simulink model "adc_behavioral"  (R2026a)
settings: Solver=FixedStepDiscrete  StartTime=0  StopTime=4095  FixedStep=1
model workspace (MAT data in the model file):
  C : object (value not decoded)
  d1_signal = [0 1 2 3 4 5 6 7 8 9 10 11 ... (8192 elements, 4096x2)]
  d2_signal = [0 1 2 3 4 5 6 7 8 9 10 11 ... (8192 elements, 4096x2)]
  n_signal = [0 1 2 3 4 5 6 7 8 9 10 11 ... (8192 elements, 4096x2)]
  x_signal = [0 1 2 3 4 5 6 7 8 9 10 11 ... (8192 elements, 4096x2)]
values from neighbouring files (symbols this model uses):
  C = entry.parameters    [adc_load_case.m]    (also in audit_adc_model.m = evalin(workspace,'C'))
(part 2 of 2)

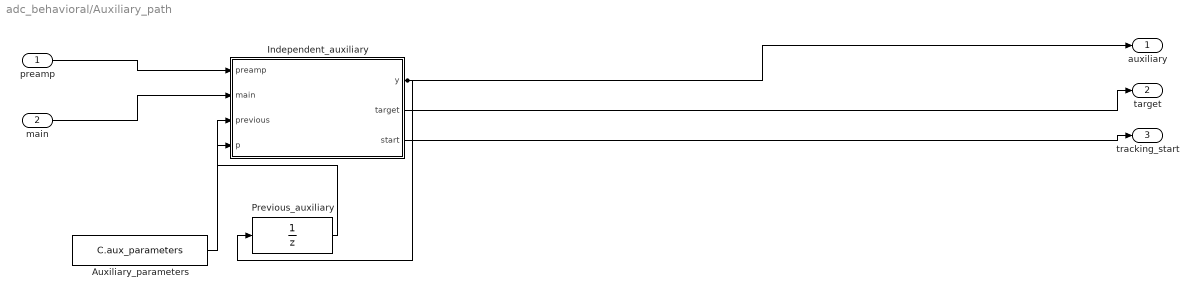
== system adc_behavioral/Auxiliary_path ==
  preamp : Inport
  main : Inport  Port=2
  Auxiliary_parameters : Constant  Value=C.aux_parameters  SampleTime=1
  Independent_auxiliary : MATLAB Function  TreatAsAtomicUnit=on
  Previous_auxiliary : UnitDelay  InitialCondition=C.initial_analog(2)
  auxiliary : Outport
  target : Outport  Port=2
  tracking_start : Outport  Port=3
  wires:
  preamp/1 -> Independent_auxiliary/1(preamp)
  main/1 -> Independent_auxiliary/2(main)
  Previous_auxiliary/1 -> Independent_auxiliary/3(previous)
  Auxiliary_parameters/1 -> Independent_auxiliary/4(p)
  Independent_auxiliary/1(y) -> Previous_auxiliary/1, auxiliary/1
  Independent_auxiliary/2(target) -> target/1
  Independent_auxiliary/3(start) -> tracking_start/1

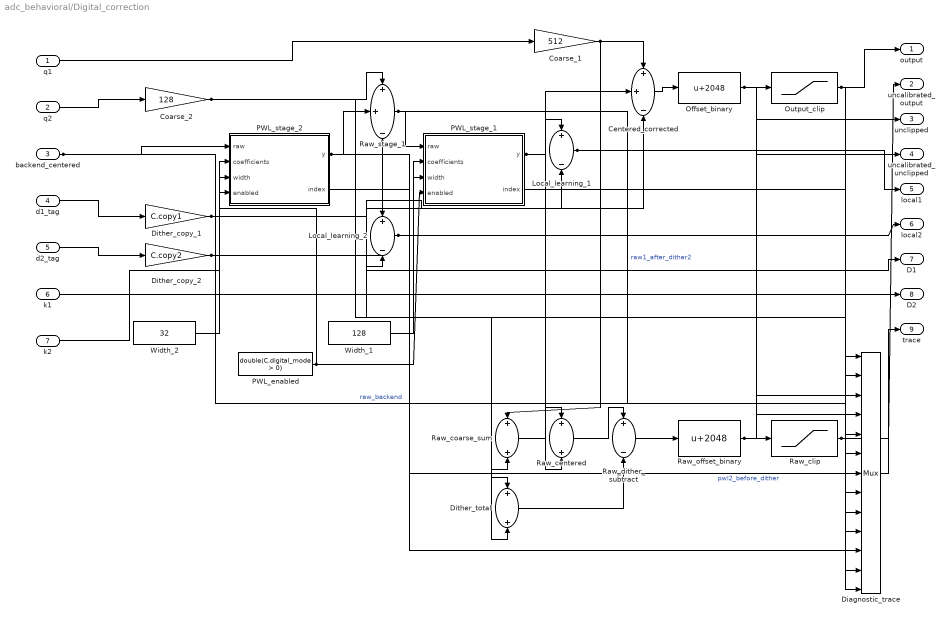
== system adc_behavioral/Digital_correction ==
  q1 : Inport
  q2 : Inport  Port=2
  backend_centered : Inport  Port=3
  d1_tag : Inport  Port=4
  d2_tag : Inport  Port=5
  k1 : Inport  Port=6
  k2 : Inport  Port=7
  Centered_corrected : Sum  Inputs=++-
  Coarse_1 : Gain  Gain=512
  Coarse_2 : Gain  Gain=128
  Diagnostic_trace : Mux  Inputs=13
  Dither_copy_1 : Gain  Gain=C.copy1
  Dither_copy_2 : Gain  Gain=C.copy2
  Dither_total : Sum
  Local_learning_1 : Sum  Inputs=+-
  Local_learning_2 : Sum  Inputs=+-
  Offset_binary : Bias  Bias=2048  SaturateOnIntegerOverflow=off
  Output_clip : Saturate  UpperLimit=4095  LowerLimit=0
  PWL_enabled : Constant  Value=double(C.digital_mode > 0)  SampleTime=1
  PWL_stage_1 : MATLAB Function  TreatAsAtomicUnit=on
  PWL_stage_2 : MATLAB Function  TreatAsAtomicUnit=on
  Raw_centered : Sum
  Raw_clip : Saturate  UpperLimit=4095  LowerLimit=0
  Raw_coarse_sum : Sum
  Raw_dither_subtract : Sum  Inputs=+-
  Raw_offset_binary : Bias  Bias=2048  SaturateOnIntegerOverflow=off
  Raw_stage_1 : Sum  Inputs=++-
  Width_1 : Constant  Value=128  SampleTime=1
  Width_2 : Constant  Value=32  SampleTime=1
  output : Outport
  uncalibrated_output : Outport  Port=2
  unclipped : Outport  Port=3
  uncalibrated_unclipped : Outport  Port=4
  local1 : Outport  Port=5
  local2 : Outport  Port=6
  D1 : Outport  Port=7
  D2 : Outport  Port=8
  trace : Outport  Port=9
  wires:
  d1_tag/1 -> Dither_copy_1/1
  d2_tag/1 -> Dither_copy_2/1
  q1/1 -> Coarse_1/1
  q2/1 -> Coarse_2/1
  backend_centered/1 -> PWL_stage_2/1(raw), Raw_centered/2  "raw_backend"
  k2/1 -> PWL_stage_2/2(coefficients)
  Width_2/1 -> PWL_stage_2/3(width)
  PWL_enabled/1 -> PWL_stage_2/4(enabled), PWL_stage_1/4(enabled)
  Coarse_2/1 -> Raw_stage_1/1, Raw_coarse_sum/2
  PWL_stage_2/1(y) -> Raw_stage_1/2, Local_learning_2/1, Diagnostic_trace/7  "pwl2_before_dither"
  Dither_copy_2/1 -> Raw_stage_1/3, Local_learning_2/2, Dither_total/2, D2/1, Diagnostic_trace/13
  Raw_stage_1/1 -> PWL_stage_1/1(raw), Diagnostic_trace/5  "raw1_after_dither2"
  k1/1 -> PWL_stage_1/2(coefficients)
  Width_1/1 -> PWL_stage_1/3(width)
  PWL_stage_1/1(y) -> Local_learning_1/1, Centered_corrected/2, Diagnostic_trace/6
  Dither_copy_1/1 -> Local_learning_1/2, Centered_corrected/3, Dither_total/1, D1/1, Diagnostic_trace/12
  Coarse_1/1 -> Centered_corrected/1, Raw_coarse_sum/1
  Centered_corrected/1 -> Offset_binary/1
  Offset_binary/1 -> Output_clip/1, unclipped/1, Diagnostic_trace/3
  Raw_coarse_sum/1 -> Raw_centered/1
  Raw_centered/1 -> Raw_dither_subtract/1
  Dither_total/1 -> Raw_dither_subtract/2
  Raw_dither_subtract/1 -> Raw_offset_binary/1
  Raw_offset_binary/1 -> Raw_clip/1, uncalibrated_unclipped/1, Diagnostic_trace/4
  Output_clip/1 -> output/1, Diagnostic_trace/1
  Raw_clip/1 -> uncalibrated_output/1, Diagnostic_trace/2
  Local_learning_1/1 -> local1/1, Diagnostic_trace/8
  Local_learning_2/1 -> local2/1, Diagnostic_trace/9
  PWL_stage_1/2(index) -> Diagnostic_trace/10
  PWL_stage_2/2(index) -> Diagnostic_trace/11
  Diagnostic_trace/1 -> trace/1

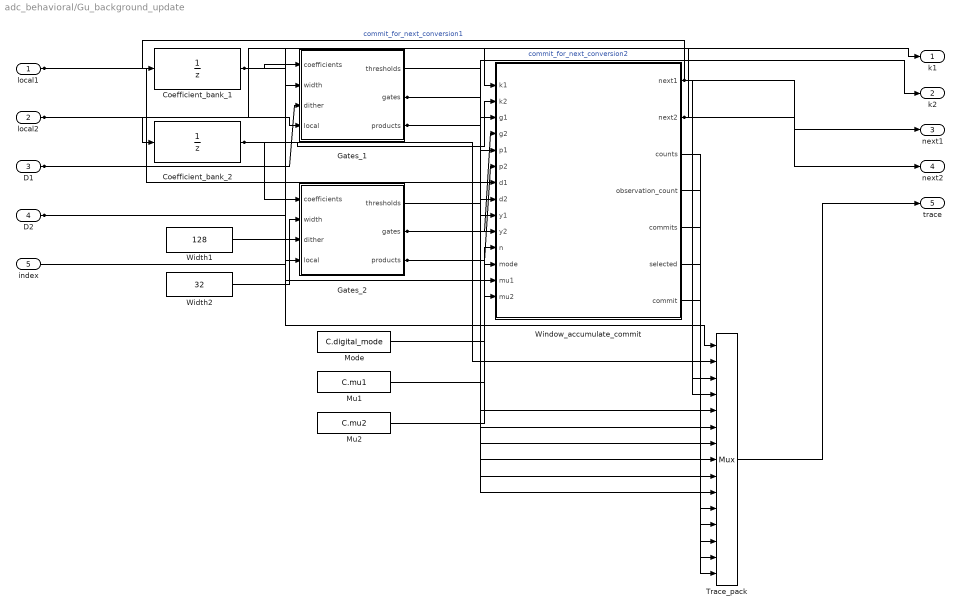
== system adc_behavioral/Gu_background_update ==
  local1 : Inport
  local2 : Inport  Port=2
  D1 : Inport  Port=3
  D2 : Inport  Port=4
  index : Inport  Port=5
  Coefficient_bank_1 : UnitDelay  InitialCondition=C.initial1
  Coefficient_bank_2 : UnitDelay  InitialCondition=C.initial2
  Gates_1 : MATLAB Function  TreatAsAtomicUnit=on
  Gates_2 : MATLAB Function  TreatAsAtomicUnit=on
  Mode : Constant  Value=C.digital_mode  SampleTime=1
  Mu1 : Constant  Value=C.mu1  SampleTime=1
  Mu2 : Constant  Value=C.mu2  SampleTime=1
  Trace_pack : Mux  Inputs=15
  Width1 : Constant  Value=128  SampleTime=1
  Width2 : Constant  Value=32  SampleTime=1
  Window_accumulate_commit : MATLAB Function  TreatAsAtomicUnit=on
  k1 : Outport
  k2 : Outport  Port=2
  next1 : Outport  Port=3
  next2 : Outport  Port=4
  trace : Outport  Port=5
  wires:
  Coefficient_bank_1/1 -> Gates_1/1(coefficients), Window_accumulate_commit/1(k1), k1/1, Trace_pack/1
  Coefficient_bank_2/1 -> Gates_2/1(coefficients), Window_accumulate_commit/2(k2), k2/1, Trace_pack/2
  Width1/1 -> Gates_1/2(width)
  Width2/1 -> Gates_2/2(width)
  D1/1 -> Gates_1/3(dither), Window_accumulate_commit/7(d1)
  D2/1 -> Gates_2/3(dither), Window_accumulate_commit/8(d2)
  local1/1 -> Gates_1/4(local), Window_accumulate_commit/9(y1)
  local2/1 -> Gates_2/4(local), Window_accumulate_commit/10(y2)
  Gates_1/2(gates) -> Window_accumulate_commit/3(g1), Trace_pack/7
  Gates_2/2(gates) -> Window_accumulate_commit/4(g2), Trace_pack/8
  Gates_1/3(products) -> Window_accumulate_commit/5(p1), Trace_pack/9
  Gates_2/3(products) -> Window_accumulate_commit/6(p2), Trace_pack/10
  index/1 -> Window_accumulate_commit/11(n)
  Mode/1 -> Window_accumulate_commit/12(mode)
  Mu1/1 -> Window_accumulate_commit/13(mu1)
  Mu2/1 -> Window_accumulate_commit/14(mu2)
  Window_accumulate_commit/1(next1) -> Coefficient_bank_1/1, next1/1, Trace_pack/3  "commit_for_next_conversion1"
  Window_accumulate_commit/2(next2) -> Coefficient_bank_2/1, next2/1, Trace_pack/4  "commit_for_next_conversion2"
  Gates_1/1(thresholds) -> Trace_pack/5
  Gates_2/1(thresholds) -> Trace_pack/6
  Window_accumulate_commit/3(counts) -> Trace_pack/11
  Window_accumulate_commit/4(observation_count) -> Trace_pack/12
  Window_accumulate_commit/5(commits) -> Trace_pack/13
  Window_accumulate_commit/6(selected) -> Trace_pack/14
  Window_accumulate_commit/7(commit) -> Trace_pack/15
  Trace_pack/1 -> trace/1

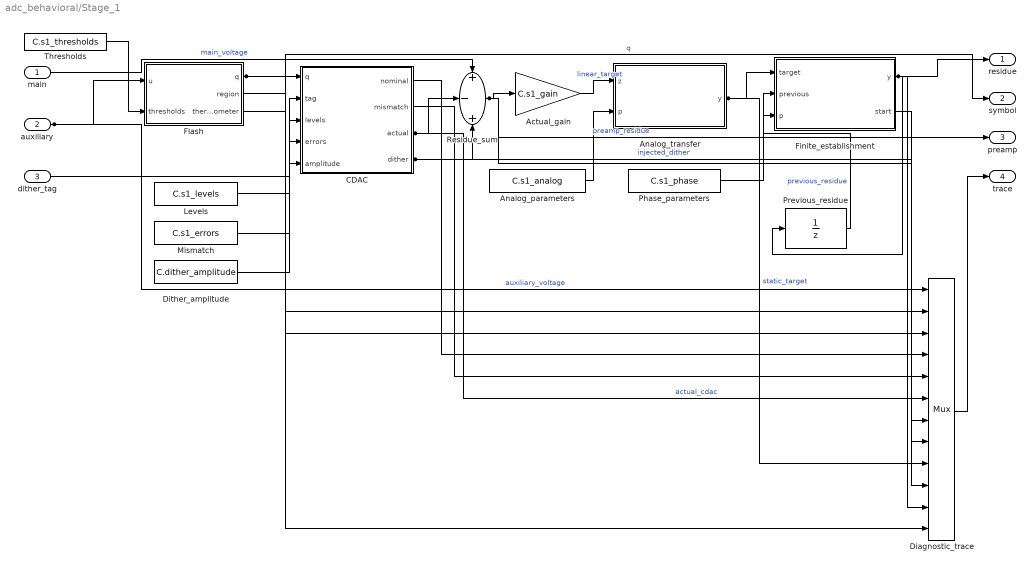
== system adc_behavioral/Stage_1 ==
  main : Inport
  auxiliary : Inport  Port=2
  dither_tag : Inport  Port=3
  Actual_gain : Gain  Gain=C.s1_gain
  Analog_parameters : Constant  Value=C.s1_analog  SampleTime=1
  Analog_transfer : MATLAB Function  TreatAsAtomicUnit=on
  CDAC : MATLAB Function  TreatAsAtomicUnit=on
  Diagnostic_trace : Mux  Inputs=12
  Dither_amplitude : Constant  Value=C.dither_amplitude  SampleTime=1
  Finite_establishment : MATLAB Function  TreatAsAtomicUnit=on
  Flash : MATLAB Function  TreatAsAtomicUnit=on
  Levels : Constant  Value=C.s1_levels  SampleTime=1
  Mismatch : Constant  Value=C.s1_errors  SampleTime=1
  Phase_parameters : Constant  Value=C.s1_phase  SampleTime=1
  Previous_residue : UnitDelay  InitialCondition=C.initial_analog(1)
  Residue_sum : Sum  Inputs=+-+
  Thresholds : Constant  Value=C.s1_thresholds  SampleTime=1
  residue : Outport
  symbol : Outport  Port=2
  preamp : Outport  Port=3
  trace : Outport  Port=4
  wires:
  auxiliary/1 -> Flash/1(u), Diagnostic_trace/1  "auxiliary_voltage"
  Thresholds/1 -> Flash/2(thresholds)
  Flash/1(q) -> CDAC/1(q), symbol/1, Diagnostic_trace/2  "q"
  dither_tag/1 -> CDAC/2(tag)
  Levels/1 -> CDAC/3(levels)
  Mismatch/1 -> CDAC/4(errors)
  Dither_amplitude/1 -> CDAC/5(amplitude)
  main/1 -> Residue_sum/1  "main_voltage"
  CDAC/3(actual) -> Residue_sum/2, Diagnostic_trace/6  "actual_cdac"
  CDAC/4(dither) -> Residue_sum/3, Diagnostic_trace/7  "injected_dither"
  Residue_sum/1 -> Actual_gain/1, preamp/1, Diagnostic_trace/8  "preamp_residue"
  Actual_gain/1 -> Analog_transfer/1(z)  "linear_target"
  Analog_parameters/1 -> Analog_transfer/2(p)
  Analog_transfer/1(y) -> Finite_establishment/1(target), Diagnostic_trace/9  "static_target"
  Previous_residue/1 -> Finite_establishment/2(previous)  "previous_residue"
  Phase_parameters/1 -> Finite_establishment/3(p)
  Finite_establishment/1(y) -> Previous_residue/1, residue/1, Diagnostic_trace/11
  Flash/2(region) -> Diagnostic_trace/3
  CDAC/1(nominal) -> Diagnostic_trace/4
  CDAC/2(mismatch) -> Diagnostic_trace/5
  Finite_establishment/2(start) -> Diagnostic_trace/10
  Flash/3(thermometer) -> Diagnostic_trace/12
  Diagnostic_trace/1 -> trace/1

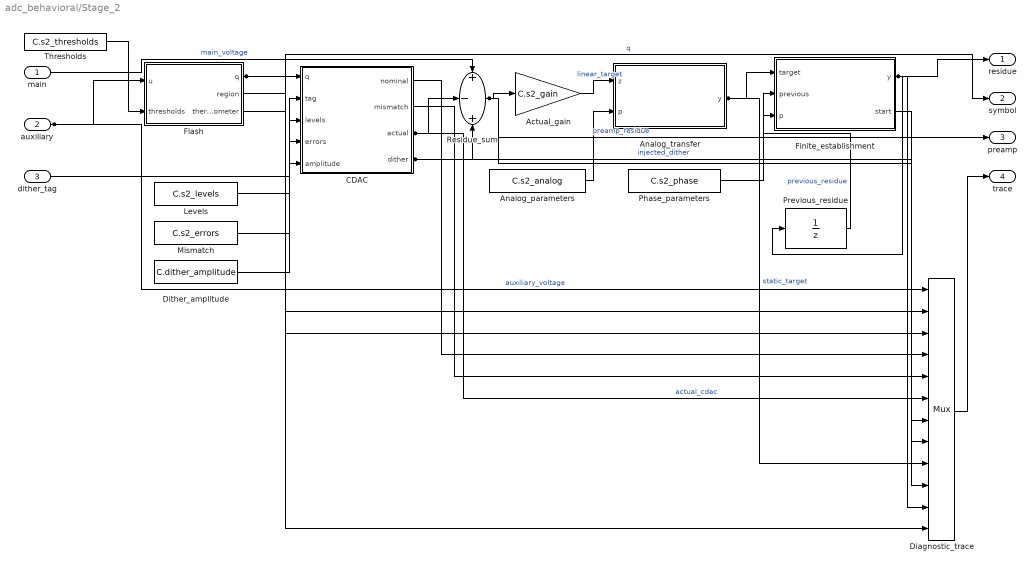
== system adc_behavioral/Stage_2 ==
  main : Inport
  auxiliary : Inport  Port=2
  dither_tag : Inport  Port=3
  Actual_gain : Gain  Gain=C.s2_gain
  Analog_parameters : Constant  Value=C.s2_analog  SampleTime=1
  Analog_transfer : MATLAB Function  TreatAsAtomicUnit=on
  CDAC : MATLAB Function  TreatAsAtomicUnit=on
  Diagnostic_trace : Mux  Inputs=12
  Dither_amplitude : Constant  Value=C.dither_amplitude  SampleTime=1
  Finite_establishment : MATLAB Function  TreatAsAtomicUnit=on
  Flash : MATLAB Function  TreatAsAtomicUnit=on
  Levels : Constant  Value=C.s2_levels  SampleTime=1
  Mismatch : Constant  Value=C.s2_errors  SampleTime=1
  Phase_parameters : Constant  Value=C.s2_phase  SampleTime=1
  Previous_residue : UnitDelay  InitialCondition=C.initial_analog(3)
  Residue_sum : Sum  Inputs=+-+
  Thresholds : Constant  Value=C.s2_thresholds  SampleTime=1
  residue : Outport
  symbol : Outport  Port=2
  preamp : Outport  Port=3
  trace : Outport  Port=4
  wires:
  auxiliary/1 -> Flash/1(u), Diagnostic_trace/1  "auxiliary_voltage"
  Thresholds/1 -> Flash/2(thresholds)
  Flash/1(q) -> CDAC/1(q), symbol/1, Diagnostic_trace/2  "q"
  dither_tag/1 -> CDAC/2(tag)
  Levels/1 -> CDAC/3(levels)
  Mismatch/1 -> CDAC/4(errors)
  Dither_amplitude/1 -> CDAC/5(amplitude)
  main/1 -> Residue_sum/1  "main_voltage"
  CDAC/3(actual) -> Residue_sum/2, Diagnostic_trace/6  "actual_cdac"
  CDAC/4(dither) -> Residue_sum/3, Diagnostic_trace/7  "injected_dither"
  Residue_sum/1 -> Actual_gain/1, preamp/1, Diagnostic_trace/8  "preamp_residue"
  Actual_gain/1 -> Analog_transfer/1(z)  "linear_target"
  Analog_parameters/1 -> Analog_transfer/2(p)
  Analog_transfer/1(y) -> Finite_establishment/1(target), Diagnostic_trace/9  "static_target"
  Previous_residue/1 -> Finite_establishment/2(previous)  "previous_residue"
  Phase_parameters/1 -> Finite_establishment/3(p)
  Finite_establishment/1(y) -> Previous_residue/1, residue/1, Diagnostic_trace/11
  Flash/2(region) -> Diagnostic_trace/3
  CDAC/1(nominal) -> Diagnostic_trace/4
  CDAC/2(mismatch) -> Diagnostic_trace/5
  Finite_establishment/2(start) -> Diagnostic_trace/10
  Flash/3(thermometer) -> Diagnostic_trace/12
  Diagnostic_trace/1 -> trace/1

== matlab function adc_behavioral/Stage_2/Analog_transfer ==
  data: z input; y output; p input
function y = adc_analog(z,p)
%#codegen
% z = actual_gain * residue_preamp. p: mode,a,b,domain,ideal5,distorted5.
mode = p(1);
if mode == 0
    y = z;
elseif mode == 1
    assert(abs(z) <= p(4));
    y = p(2)*z + p(3)*z^3;
else
    magnitude = abs(z);
    assert(magnitude <= p(9));
    index = 1;
    for j=2:5
        if magnitude >= p(4+j)
            index = j;
        end
    end
    index = min(index,4);
    slope = (p(10+index)-p(9+index))/(p(5+index)-p(4+index));
    y = sign(z)*(p(9+index)+slope*(magnitude-p(4+index)));
end
end

== matlab function adc_behavioral/Stage_2/Finite_establishment ==
  data: target input; y output; previous input; p input; start output
function [y,start] = adc_settle(target,previous,p)
%#codegen
% mode0 static; mode1/2 one-phase; mode3 tracking+amplification.
if p(1) == 0
    start = 0;
    y = target;
elseif p(1) == 3
    start = p(4) + p(3)*(previous-p(4));
    y = target + p(2)*(start-target);
else
    start = previous;
    y = (1-p(2))*target + p(2)*previous;
end
end

== matlab function adc_behavioral/SAR_8bit ==
  data: u input; raw output; n input; centered output; channel output; quantized output
function [raw,centered,channel,quantized] = adc_sar(u,n)
%#codegen
% Preserve Python's (u-low)/step order at floating boundary neighbors.
raw = min(max(floor((u-(-1))/(2/256)),0),255);
centered = raw-128;
channel = mod(n,4);
quantized = -1+(raw+0.5)*(2/256);
end

== matlab function adc_behavioral/Digital_correction/PWL_stage_2 ==
  data: raw input; y output; coefficients input; width input; enabled input; index output
function [y,index] = adc_pwl(raw,coefficients,width,enabled)
%#codegen
if enabled == 0
    y = raw;
    index = -1;
    return
end
assert(raw >= -4*width && raw < 4*width);
magnitude = abs(raw);
index = min(floor(magnitude/width),3);
local = magnitude-index*width;
offset = 0;
for j=1:4
    if j <= index
        offset = offset+width*coefficients(j);
    end
end
y = sign(raw)*(offset+coefficients(index+1)*local);
end

== matlab function adc_behavioral/Digital_correction/PWL_stage_1 ==
  data: raw input; y output; coefficients input; width input; enabled input; index output
function [y,index] = adc_pwl(raw,coefficients,width,enabled)
%#codegen
if enabled == 0
    y = raw;
    index = -1;
    return
end
assert(raw >= -4*width && raw < 4*width);
magnitude = abs(raw);
index = min(floor(magnitude/width),3);
local = magnitude-index*width;
offset = 0;
for j=1:4
    if j <= index
        offset = offset+width*coefficients(j);
    end
end
y = sign(raw)*(offset+coefficients(index+1)*local);
end

== matlab function adc_behavioral/Gu_background_update/Gates_1 ==
  data: coefficients input; thresholds output; width input; dither input; local input; gates output; products output
function [thresholds,gates,products] = adc_gate(coefficients,width,dither,local)
%#codegen
thresholds = zeros(1,4);
gates = ones(1,4);
products = zeros(1,4);
cumulative = 0;
for j=1:4
    if j > 1
        cumulative = cumulative+width*coefficients(j-1);
        thresholds(j) = cumulative;
        gates(j) = double(abs(local) >= cumulative);
    end
    if gates(j) == 1
        products(j) = dither*local;
    end
end
end

== matlab function adc_behavioral/Gu_background_update/Gates_2 ==
  data: coefficients input; thresholds output; width input; dither input; local input; gates output; products output
function [thresholds,gates,products] = adc_gate(coefficients,width,dither,local)
%#codegen
thresholds = zeros(1,4);
gates = ones(1,4);
products = zeros(1,4);
cumulative = 0;
for j=1:4
    if j > 1
        cumulative = cumulative+width*coefficients(j-1);
        thresholds(j) = cumulative;
        gates(j) = double(abs(local) >= cumulative);
    end
    if gates(j) == 1
        products(j) = dither*local;
    end
end
end

== matlab function adc_behavioral/Gu_background_update/Window_accumulate_commit ==
  data: k1 input; next1 output; k2 input; g1 input; g2 input; p1 input; p2 input; d1 input; d2 input; y1 input; y2 input; n input; mode input; mu1 input; mu2 input; next2 output; counts output; observation_count output; commits output; selected output; commit output
function [next1,next2,counts,observation_count,commits,selected,commit] = adc_update(k1,k2,g1,g2,p1,p2,d1,d2,y1,y2,n,mode,mu1,mu2)
%#codegen
% Window accumulators only; visible coefficient memory is in Unit Delays.
persistent sums gate_counts observations commit_count
if isempty(sums)
    sums = zeros(1,8);
    gate_counts = zeros(1,8);
    observations = 0;
    commit_count = 0;
end
next1=k1;
next2=k2;
selected=0;
commit=0;
position=mod(n,120);
if mode == 2
    selected=1;
elseif mode == 3
    selected=double(position < 4);
elseif mode == 4
    selected=1;
end
if selected == 1
    observations=observations+1;
    gate_counts=gate_counts+[g1 g2];
    if mode == 2
        for j=1:4
            if g1(j) == 1
                next1(j)=min(max(k1(j)-mu1(j)*d1*y1,0),2);
            end
            if g2(j) == 1
                next2(j)=min(max(k2(j)-mu2(j)*d2*y2,0),2);
            end
        end
        commit=1;
    else
        sums=sums+[p1 p2];
    end
end
if (mode == 3 || mode == 4) && position == 119
    if mode == 3
        number=4;
        multiplier=30;
    else
        number=120;
        multiplier=1;
    end
    for j=1:4
        % Same order as original update_block_mean(adapted mu).
        next1(j)=min(max(k1(j)-(mu1(j)*multiplier*number)*(sums(j)/number),0),2);
        next2(j)=min(max(k2(j)-(mu2(j)*multiplier*number)*(sums(j+4)/number),0),2);
    end
    sums=zeros(1,8);
    commit=1;
end
commit_count=commit_count+commit;
counts=gate_counts;
observation_count=observations;
commits=commit_count;
end

== matlab function adc_behavioral/Overload_and_clipping ==
  data: x input; flags output; aux1 input; r1 input; aux2 input; r2 input; raw_unclipped input; corrected_unclipped input
function flags = adc_flags(x,aux1,r1,aux2,r2,raw_unclipped,corrected_unclipped)
%#codegen
% Every overload/clipping event is retained; auxiliary alone loses no data.
flags=zeros(1,17);
flags(1)=double(x < -1); flags(2)=double(x >= 1);
flags(3)=double(aux1 < -1); flags(4)=double(aux1 >= 1);
flags(5)=double(r1 < -1); flags(6)=double(r1 >= 1);
flags(7)=double(aux2 < -1); flags(8)=double(aux2 >= 1);
flags(9)=double(r2 < -1); flags(10)=double(r2 >= 1);
flags(11)=double(raw_unclipped < 0); flags(12)=double(raw_unclipped > 4095);
flags(13)=double(corrected_unclipped < 0); flags(14)=double(corrected_unclipped > 4095);
physical=any(flags([1 2 5 6 9 10]));
flags(15)=double(~physical && ~any(flags(11:12)));
flags(16)=double(~any(flags(13:14)));
flags(17)=double(~physical && ~any(flags(13:14)));
end

== matlab function adc_behavioral/Stage_1/CDAC ==
  data: q input; nominal output; tag input; levels input; errors input; amplitude input; mismatch output; actual output; dither output
function [nominal,mismatch,actual,dither] = adc_cdac(q,tag,levels,errors,amplitude)
%#codegen
nominal = levels(q+5);
mismatch = errors(q+5);
actual = nominal + mismatch;
dither = tag * amplitude; % tag=0 represents Python None (disabled).
end

== matlab function adc_behavioral/Stage_1/Flash ==
  data: u input; q output; thresholds input; region output; thermometer output
function [q,region,thermometer] = adc_flash(u,thresholds)
%#codegen
% Python bisect_right: equality belongs to the higher region.
thermometer = zeros(1,8);
region = 0;
for j=1:8
    thermometer(j) = double(u >= thresholds(j));
    region = region + thermometer(j);
end
q = region - 4;
end

== matlab function adc_behavioral/Stage_1/Analog_transfer ==
  data: z input; y output; p input
function y = adc_analog(z,p)
%#codegen
% z = actual_gain * residue_preamp. p: mode,a,b,domain,ideal5,distorted5.
mode = p(1);
if mode == 0
    y = z;
elseif mode == 1
    assert(abs(z) <= p(4));
    y = p(2)*z + p(3)*z^3;
else
    magnitude = abs(z);
    assert(magnitude <= p(9));
    index = 1;
    for j=2:5
        if magnitude >= p(4+j)
            index = j;
        end
    end
    index = min(index,4);
    slope = (p(10+index)-p(9+index))/(p(5+index)-p(4+index));
    y = sign(z)*(p(9+index)+slope*(magnitude-p(4+index)));
end
end

== matlab function adc_behavioral/Stage_1/Finite_establishment ==
  data: target input; y output; previous input; p input; start output
function [y,start] = adc_settle(target,previous,p)
%#codegen
% mode0 static; mode1/2 one-phase; mode3 tracking+amplification.
if p(1) == 0
    start = 0;
    y = target;
elseif p(1) == 3
    start = p(4) + p(3)*(previous-p(4));
    y = target + p(2)*(start-target);
else
    start = previous;
    y = (1-p(2))*target + p(2)*previous;
end
end

== matlab function adc_behavioral/Auxiliary_path/Independent_auxiliary ==
  data: preamp input; y output; main input; previous input; p input; target output; start output
function [y,target,start] = adc_auxiliary(preamp,main,previous,p)
%#codegen
% p: mode,rho,offset,main_gain,aux_gain,a,b,domain,amp,track,track_target.
if p(1) == 0 || p(1) == 1
    target = p(2)*main+p(3);
    start = 0;
    y = target;
elseif p(1) == 2
    target = p(2)*p(4)*preamp+p(3);
    start = previous;
    y = (1-p(9))*target+p(9)*previous;
else
    z = p(5)*preamp;
    assert(abs(z) <= p(8));
    target = p(6)*z+p(7)*z^3;
    start = p(11)+p(10)*(previous-p(11));
    y = target+p(9)*(start-target);
end
end

== matlab function adc_behavioral/Stage_2/Flash ==
  data: u input; q output; thresholds input; region output; thermometer output
function [q,region,thermometer] = adc_flash(u,thresholds)
%#codegen
% Python bisect_right: equality belongs to the higher region.
thermometer = zeros(1,8);
region = 0;
for j=1:8
    thermometer(j) = double(u >= thresholds(j));
    region = region + thermometer(j);
end
q = region - 4;
end

== matlab function adc_behavioral/Stage_2/CDAC ==
  data: q input; nominal output; tag input; levels input; errors input; amplitude input; mismatch output; actual output; dither output
function [nominal,mismatch,actual,dither] = adc_cdac(q,tag,levels,errors,amplitude)
%#codegen
nominal = levels(q+5);
mismatch = errors(q+5);
actual = nominal + mismatch;
dither = tag * amplitude; % tag=0 represents Python None (disabled).
end
